simulink library "limo_lib_R2026a"  (R2026a)
settings: Solver=VariableStepAuto
PostLoadFcn:
  | addpath(fileparts(get_param('limo_lib', 'FileName')));
undefined symbols (not defined in the file or in its folder): limo
settings Model: Creator=jkreiss  LastModifiedBy=mattia
settings SFSimCC: SimGPUStackLimitPerThread=51200
settings RTWCC: GPUStackLimitPerThread=51200

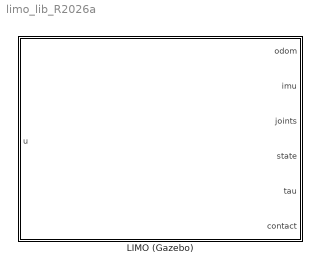
== system limo_lib_R2026a ==
  LIMO (Gazebo) : Subsystem  mask(AgileX LIMO (Gazebo)){input_mode=Steering angle: [v; gamma], pose_mode=Origin, custom_pose=[0 0 0], mu=1, v_eps=1e-3}
      mask prompts: input_mode "Input u:"; pose_mode "Initial pose:"; custom_pose "Custom pose [X (m), Y (m), psi (rad)]:"; mu "Friction coefficient mu (Gazebo: 1):"; v_eps "Friction regularisation velocity (m/s):"
      mask help:
      | AgileX LIMO with the dynamics of the ENSEM Gazebo simulation (ROS 2 Foxy, limo_car/gazebo/ackermann_with_sensor.xacro).
      |
      | Input u:
      |   Steering angle: [v (m/s); gamma (rad)], gamma = central steering angle (tan(gamma) = L/R), positive to the left, limited to 30 deg
      |   cmd_vel: [linear.x (m/s); angular.z (rad/s)] as on the ROS topic
      |   Joint efforts: [tau_FL; tau_FR; tau_RL; tau_RR; tau_delta_L; tau_delta_R] (N.m)
      |
      | Outputs: odom [X Y psi v_x v_y r], imu [q (4); omega (3); a (3)], joints [omega (4); delta (2)], state (14), tau (6), contact [F_x (4); F_y (4); F_n (4)].
      |
      | The other parameters are in limo.parameters() (+limo/parameters.m).
      mask init:
      | % Parameters of the LIMO, with the choices of the mask
      | limo_p = limo.parameters();
      | 
      | switch pose_mode
      |     case 1
      |         limo_p.initial.pose = [0; 0; 0];
      |     case 2
      |         limo_p.initial.pose = limo_p.initial.room207_pose;
      |     otherwise
      |         limo_p.initial.pose = custom_pose(:);
      | end
      | 
      | limo_p.contact.friction.mu = mu;
      | limo_p.contact.friction.regularization_velocity = v_eps;
      | 
      | % Block icon, stored next to limo_lib.slx
      | limo_icon = fullfile(fileparts(which('limo_lib')), 'images', 'limo_icon.png');
      mask Help: web(fullfile(fileparts(which('limo_lib')), 'README.md'))
      mask TypeOptions input_mode: Steering angle: [v; gamma] | cmd_vel: [v; yaw rate] (twist adapter) | Joint efforts (own controller)
      mask TypeOptions pose_mode: Origin | Room 207 spawn | Custom
      mask Callback pose_mode:
      | custom = Simulink.Mask.get(gcb).getParameter('custom_pose');
      | if strcmp(get_param(gcb, 'pose_mode'), 'Custom')
      |     custom.Enabled = 'on';
      | else
      |     custom.Enabled = 'off';
      | end
      mask DialogControl tab_command Prompt: Command
      mask DialogControl tab_pose Prompt: Initial pose
      mask DialogControl tab_contact Prompt: Contact
      mask Display:
      | image(limo_icon, [0.22 0.16 0.52 0.52]);
      | switch input_mode
      |     case 1
      |         port_label('input', 1, 'v, \gamma', 'texmode', 'on');
      |     case 2
      |         port_label('input', 1, 'cmd_vel');
      |     otherwise
      |         port_label('input', 1, 'tau');
      | end
      | port_label('output', 1, 'odom');
      | port_label('output', 2, 'imu');
      | port_label('output', 3, 'joints');
      | port_label('output', 4, 'state');
      | port_label('output', 5, 'tau');
      | port_label('output', 6, 'contact');

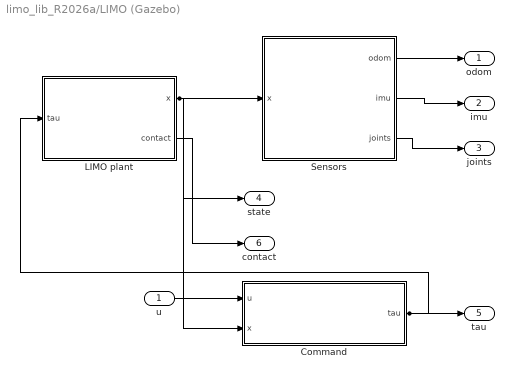
== system limo_lib_R2026a/LIMO (Gazebo) ==
  u : Inport
  Command : Subsystem  Variant=on
  LIMO plant : Subsystem
  Sensors : Subsystem
  odom : Outport
  imu : Outport  Port=2
  joints : Outport  Port=3
  state : Outport  Port=4
  tau : Outport  Port=5
  contact : Outport  Port=6
  wires:
  LIMO plant/2(contact) -> contact/1
  LIMO plant/1(x) -> Command/2(x), Sensors/1(x), state/1
  u/1 -> Command/1(u)
  Sensors/3(joints) -> joints/1
  Sensors/2(imu) -> imu/1
  Sensors/1(odom) -> odom/1
  Command/1(tau) -> tau/1, LIMO plant/1(tau)

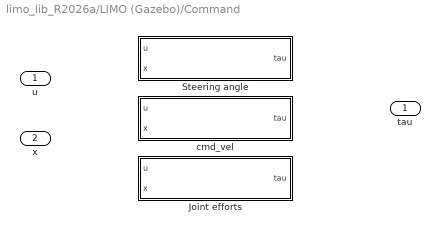
== system limo_lib_R2026a/LIMO (Gazebo)/Command ==
  u : Inport
  x : Inport  Port=2
  Joint efforts : Subsystem  VariantControl=input_mode == 3
  Steering angle : Subsystem  VariantControl=input_mode == 1
  cmd_vel : Subsystem  VariantControl=input_mode == 2
  tau : Outport

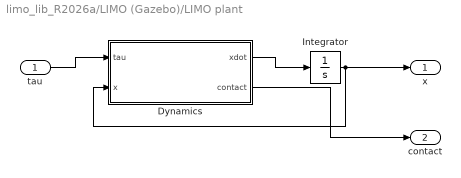
== system limo_lib_R2026a/LIMO (Gazebo)/LIMO plant ==
  tau : Inport
  Dynamics : MATLAB Function  TreatAsAtomicUnit=on
  Integrator : Integrator  InitialCondition=limo.initial_state(limo_p)
  x : Outport
  contact : Outport  Port=2
  wires:
  tau/1 -> Dynamics/1(tau)
  Dynamics/1(xdot) -> Integrator/1
  Integrator/1 -> x/1, Dynamics/2(x)
  Dynamics/2(contact) -> contact/1

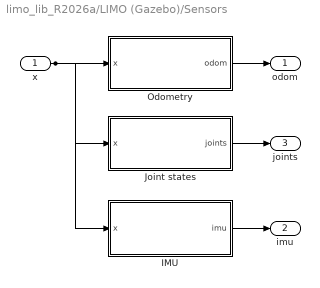
== system limo_lib_R2026a/LIMO (Gazebo)/Sensors ==
  x : Inport
  IMU : MATLAB Function  TreatAsAtomicUnit=on  SystemSampleTime=limo_p.sensors.imu.sample_time
  Joint states : MATLAB Function  TreatAsAtomicUnit=on  SystemSampleTime=limo_p.sensors.odom.sample_time
  Odometry : MATLAB Function  TreatAsAtomicUnit=on  SystemSampleTime=limo_p.sensors.odom.sample_time
  odom : Outport
  imu : Outport  Port=2
  joints : Outport  Port=3
  wires:
  IMU/1(imu) -> imu/1
  Odometry/1(odom) -> odom/1
  x/1 -> Odometry/1(x), IMU/1(x), Joint states/1(x)
  Joint states/1(joints) -> joints/1

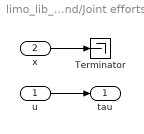
== system limo_lib_R2026a/LIMO (Gazebo)/Command/Joint efforts ==
  u : Inport
  x : Inport  Port=2
  Terminator : Terminator
  tau : Outport
  wires:
  u/1 -> tau/1
  x/1 -> Terminator/1

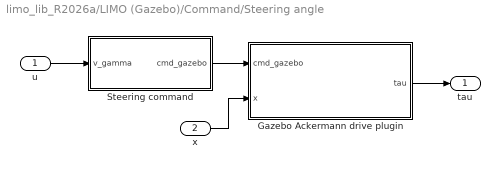
== system limo_lib_R2026a/LIMO (Gazebo)/Command/Steering angle ==
  u : Inport
  x : Inport  Port=2
  Gazebo Ackermann drive plugin : MATLAB Function  TreatAsAtomicUnit=on  SystemSampleTime=limo_p.gazebo.physics_step
  Steering command : MATLAB Function  TreatAsAtomicUnit=on
  tau : Outport
  wires:
  x/1 -> Gazebo Ackermann drive plugin/2(x)
  u/1 -> Steering command/1(v_gamma)
  Steering command/1(cmd_gazebo) -> Gazebo Ackermann drive plugin/1(cmd_gazebo)
  Gazebo Ackermann drive plugin/1(tau) -> tau/1

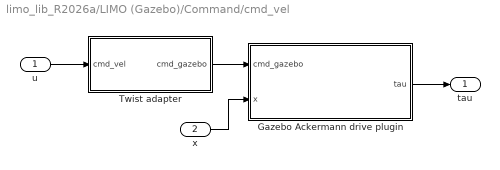
== system limo_lib_R2026a/LIMO (Gazebo)/Command/cmd_vel ==
  u : Inport
  x : Inport  Port=2
  Gazebo Ackermann drive plugin : MATLAB Function  TreatAsAtomicUnit=on  SystemSampleTime=limo_p.gazebo.physics_step
  Twist adapter : MATLAB Function  TreatAsAtomicUnit=on
  tau : Outport
  wires:
  u/1 -> Twist adapter/1(cmd_vel)
  x/1 -> Gazebo Ackermann drive plugin/2(x)
  Twist adapter/1(cmd_gazebo) -> Gazebo Ackermann drive plugin/1(cmd_gazebo)
  Gazebo Ackermann drive plugin/1(tau) -> tau/1

== matlab function limo_lib_R2026a/LIMO (Gazebo)/Command/Steering angle/Gazebo Ackermann drive plugin ==
  data: cmd_gazebo input; tau output; x input; limo_p parameter
function tau = plugin(cmd_gazebo, x, limo_p)
%PLUGIN gazebo_ros_ackermann_drive + Joint::SetForce(), run every physics step.
%
%   The plugin updates every limo_p.gazebo.plugin.sample_time and, as in
%   Gazebo, its efforts act during the next physics step only.

persistent pid step

if isempty(pid)
    pid = zeros(3, 2);
    step = 0;
end

n = round(limo_p.gazebo.plugin.sample_time/limo_p.gazebo.physics_step);

% No update at load time (no time elapsed yet)
if step > 0 && mod(step, n) == 0
    [tau_cmd, pid] = limo.gazebo_ackermann_plugin(cmd_gazebo, x([10 11 12]), pid, limo_p);
    tau = limo.gazebo_set_force(tau_cmd, x(13:14), limo_p);
else
    tau = zeros(6, 1);
end

step = step + 1;

== matlab function limo_lib_R2026a/LIMO (Gazebo)/Command/Steering angle/Steering command ==
  data: v_gamma input; cmd_gazebo output
function cmd_gazebo = steering(v_gamma)
%STEERING [v; gamma] -> /cmd_vel_gazebo (limo.gazebo_steering_command).

cmd_gazebo = limo.gazebo_steering_command(v_gamma(1), v_gamma(2));

== matlab function limo_lib_R2026a/LIMO (Gazebo)/Command/cmd_vel/Twist adapter ==
  data: cmd_vel input; cmd_gazebo output; limo_p parameter
function cmd_gazebo = adapter(cmd_vel, limo_p)
%ADAPTER /cmd_vel -> /cmd_vel_gazebo (limo.gazebo_twist_adapter).

cmd_gazebo = limo.gazebo_twist_adapter(cmd_vel(1), cmd_vel(2), limo_p);

== matlab function limo_lib_R2026a/LIMO (Gazebo)/Command/cmd_vel/Gazebo Ackermann drive plugin ==
  data: cmd_gazebo input; tau output; x input; limo_p parameter
function tau = plugin(cmd_gazebo, x, limo_p)
%PLUGIN gazebo_ros_ackermann_drive + Joint::SetForce(), run every physics step.
%
%   The plugin updates every limo_p.gazebo.plugin.sample_time and, as in
%   Gazebo, its efforts act during the next physics step only.

persistent pid step

if isempty(pid)
    pid = zeros(3, 2);
    step = 0;
end

n = round(limo_p.gazebo.plugin.sample_time/limo_p.gazebo.physics_step);

% No update at load time (no time elapsed yet)
if step > 0 && mod(step, n) == 0
    [tau_cmd, pid] = limo.gazebo_ackermann_plugin(cmd_gazebo, x([10 11 12]), pid, limo_p);
    tau = limo.gazebo_set_force(tau_cmd, x(13:14), limo_p);
else
    tau = zeros(6, 1);
end

step = step + 1;

== matlab function limo_lib_R2026a/LIMO (Gazebo)/LIMO plant/Dynamics ==
  data: tau input; xdot output; x input; contact output; limo_p parameter
function [xdot, contact] = dynamics(tau, x, limo_p)
%DYNAMICS State derivative of the LIMO (limo.plant_dynamics).
%
%   contact = [F_x (4); F_y (4); F_n (4)] in the wheel frames [N],
%   wheel order FL, FR, RL, RR.

[xdot, aux] = limo.plant_dynamics(x, tau, limo_p);

contact = [aux.F_x; aux.F_y; aux.F_n];

== matlab function limo_lib_R2026a/LIMO (Gazebo)/Sensors/Odometry ==
  data: x input; odom output
function odom = odometry(x)
%ODOMETRY Ground-truth odometry published by the Ackermann plugin.
%   odom = [X; Y; psi; v_x; v_y; r] of base_link

odom = x(1:6);

== matlab function limo_lib_R2026a/LIMO (Gazebo)/Sensors/IMU ==
  data: x input; imu output; limo_p parameter
function imu = imu_sensor(x, limo_p)
%IMU_SENSOR Gazebo IMU (limo.imu_gazebo).
%   imu = [q_x; q_y; q_z; q_w; omega (3); a (3)]

persistent v_last

if isempty(v_last)
    % Seeded with the velocity at load time
    v_last = [cos(x(3))*x(4) - sin(x(3))*x(5); sin(x(3))*x(4) + cos(x(3))*x(5)];
end

[imu, v_last] = limo.imu_gazebo(x, v_last, limo_p);

== matlab function limo_lib_R2026a/LIMO (Gazebo)/Sensors/Joint states ==
  data: x input; joints output
function joints = joint_states(x)
%JOINT_STATES Wheel rates and steering angles.
%   joints = [omega_FL; omega_FR; omega_RL; omega_RR; delta_L; delta_R]

joints = x(7:12);
